simulink model "Template_v5_0_0_2026a_Original"  (R2026a)
settings: Solver=ode4  StopTime=tsim  FixedStep=baseRate  RelTol=1e-6  AbsTol=1e-6
undefined symbols (not defined in the file or in its folder): baseRate, dataRate, DiscIntNeverNeededParam, F_thrusters_BLACK, F_thrusters_BLUE, F_thrusters_RED, home_states_BLACK, home_states_BLUE, home_states_RED, IBLACK, IBLUE, init_states_BLACK, init_states_BLUE, init_states_RED, IRED, K_BLACK, K_BLUE, K_RED, labConsoleIP, mBLACK, mBLUE, mRED, Phase0_End, Phase1_End, Phase2_End, Phase3_End, Phase3_SubPhase1_End, Phase3_SubPhase2_End, Phase3_SubPhase3_End, Phase3_SubPhase4_End, Phase4_End, Phase5_End, platformSelection, PWMFreq, serverRate, simMode, tableDamping_BLACK, tableDamping_BLUE, tableDamping_RED, tableSlope, thrust_decay_BLACK, thrust_decay_BLUE, thrust_decay_RED, thruster_dist2CG_BLACK, thruster_dist2CG_BLUE, thruster_dist2CG_RED, xLength, yLength
libraries: simulink x18, dspinverses x3, nvidiaCommlib x1
(part 1 of 7)
settings Model: Creator=SPOT  LastModifiedBy=alexandercrain
settings OptimizationCC: MaxStackSize=200000
settings HardwareCC: ProdBitPerLong=64.0  ProdLargestAtomicInteger=LongLong  ProdLargestAtomicFloat=Double  ProdHWDeviceType=ARM Compatible->ARM Cortex-A (64-bit)
settings RTWCC: SystemTargetFile=ert.tlc  HardwareBoard=NVIDIA Jetson  TLCOptions="-aInlineSetEventsForThisBaseRateFcn=TLC_FALSE -aSuppressMultiTaskScheduler=TLC_FALSE  -aRateBasedStepFcn=0"  TargetLang=C++  Description=Embedded Coder
settings ERTTargetCC: ExtModeTransport=2.0  DynamicArrayContainerType=coder::array  SupportContinuousTime=on  SupportVariableSizeSignals=on
settings SimscapeCC: SimscapeNominalValues="[{\"value\":\"1\",\"unit\":\"A\"},{\"value\":\"1\",\"unit\":\"bar\"},{\"value\":\"1\",\"unit\":\"cm^2\"},{\"value\":\"1\",\"unit\":\"cm^3/s\"},{\"value\":\"1\",\"unit\":\"kJ/kg\"},{\"value\":\"1\",\"unit\":\"kW\"},{\"value\":\"1\",\"unit\":\"l\"},{\"value\":\"1\",\"unit\":\"N\"},{\"value\":\"1\",\"unit\":\"N*m\"},{\"value\":\"1\",\"unit\":\"V\"}]"  SimscapeLogType=none  SimscapeLogDataHistory=5000.0

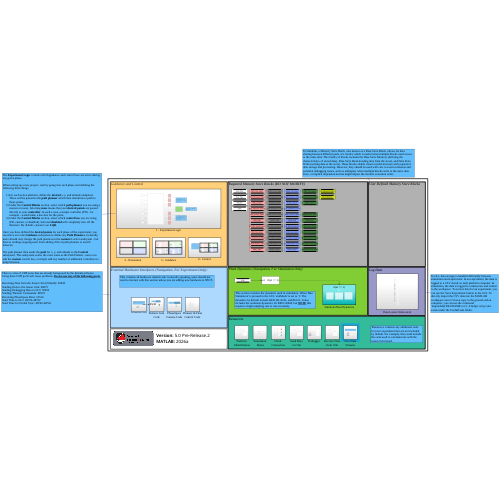
[thumbnail: Simulink's stored preview of the top-level diagram]
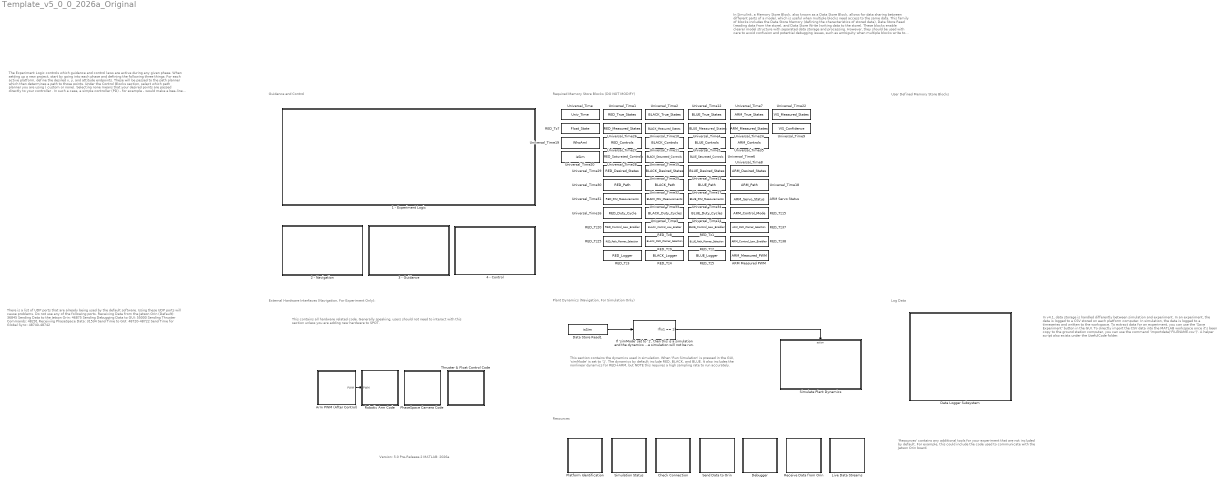
== system Template_v5_0_0_2026a_Original ==
  note: Version: 5.0 Pre-Release.2
      | MATLAB: 2026a
  note: Required Memory Store Blocks (DO NOT MODIFY)
  note: In Simulink, a Memory Store Block, also known as a Data Store Block, allows for data sharing between different parts of a model, which is useful when multiple blocks need access to the same data. This family of blocks includes the Data Store Memory (defining the characteristics of stored data), Data Store Read (reading data from the store), and Data Store Write (writing data to the store). These blocks enable clearer model structure with separated data storage and processing. However, they should be used with care to avoid confusion and potential debugging issues, such as ambiguity when multiple blocks write to the same data store, or implicit dependencies that might impact the model's execution order.
  note: User Defined Memory Store Blocks
  note: Log Data
  note: In v4.1, data storage is handled differently between simulation and experiment. In an experiment, the data is logged to a CSV stored on each platform computer. In simulation, the data is logged to a timeseries and written to the workspace. To extract data for an experiment, you can use the 'Save Experiment' button in the GUI. To directly import the CSV data into the MATLAB workspace once it's been copy to the ground station computer, you can use the command 'importdata('FILENAME.csv')'. A helper script also exists under the UsefulCode folder.
  note: Resources
  note: 'Resources' contains any additional tools for your experiment that are not included by default. For example, this could include the code used to communicate with the Jetson Orin board.
  note: Plant Dynamics (Navigation, For Simulation Only)
  note: This section contains the dynamics used in simulation. When 'Run Simulation' is pressed in the GUI, 'simMode' is set to '1'. The dynamics by default include RED, BLACK, and BLUE. It also includes the nonlinear dynamics for RED+ARM, but NOTE this requires a high sampling rate to run accurately.
  note: External Hardware Interfaces (Navigation, For Experiment Only):
  note: This contains all hardware related code. Generally speaking, users should not need to interact with this section unless you are adding new hardware to SPOT.
  note: Guidance and Control
  note: The Experiment Logic controls which guidance and control laws are active during any given phase.
      |
      | When setting up a new project, start by going into each phase and defining the following three things:
      |
      | For each active platform, define the desired x, y, and attitude endpoints. These will be passed to the path planner which then determines a path to those points.
      | Under the Control Blocks section, select which path planner you are using ( custom or none). Selecting none means that your desired points are passed directly to your controller . In such a case, a simple controller (PD) - for example - would make a bee-line for the point.
      | Under the Control Blocks section, select which control law you are using (PD, custom, or disabled). Selected disabled will completely turn off the thrusters. By default, custom is an LQR .
      |
      | Once you have defined the desired points for each phase of the experiment, you can move on to the Guidance subsystem to define any Path Planners. Generally, users should only change the path planners in the custom if-action subsytem - but there is nothing stopping users from adding 100s of path planners to switch between.
      |
      | The path planner then sends the path for x, y, and attitude to the Control subsystem. This subsystem works the exact same as the Path Planner - users can edit the custom control law, or simply add any number of additional controllers to jump between.
  note: There is a list of UDP ports that are already being used by the default software. Using these UDP ports will cause problems. Do not use any of the following ports.
      |
      | Receiving Data from the Jetson Orin (Default): 36845
      | Sending Data to the Jetson Orin: 46875
      | Sending Debugging Data to GUI: 55000
      | Sending Thruster Commands: 48291
      | Receiving PhaseSpace Data: 31534
      | Send Time to GUI: 48720-48722
      | Send Time for Global Sync: 48740-48742
  1 - Experiment Logic : Subsystem  Priority=30  TreatAsAtomicUnit=on
  2 - Navigation : Subsystem  Priority=40  TreatAsAtomicUnit=on
  3 - Guidance : Subsystem  Priority=40  TreatAsAtomicUnit=on
  4 - Control : Subsystem  Priority=50  TreatAsAtomicUnit=on
  ARM Measured PWM : DataStoreMemory  Description=ARM_Measured_PWM: the PWM each arm servo applies (its Present PWM, 885 = 100 % of the supply), written each step by the Dynamixel Arm (PWM) block on the hardware and by the RED + ARM Plant in simulation.  DataStoreName=ARM_Measured_PWM  WriteAfterWriteMsg=warning  InitialValue=[0;0;0]  ShowAdditionalParam=off
  ARM Servo Status : DataStoreMemory  Description="ARM_Controls: The simulated plant reads it at the start of each step, like the measurements, before the thruster code writes this step's command: the previous command acts for one step. (A loop through data stores needs one such step; with the plant first, the controllers get this step's measurements, as in experiments.) Before the first write, its initial value. (so its \"read before write\" and \"write after read\" checks are off)."  DataStoreName=ARM_Servo_Status  WriteAfterWriteMsg=warning  InitialValue=zeros(5,1)  ShowAdditionalParam=off
  Arm PWM (After Control) : Subsystem  Priority=61  TreatAsAtomicUnit=on
  Check Connection : Subsystem  Priority=71  TreatAsAtomicUnit=on
  Data Logger Subsystem : Subsystem  Priority=80  TreatAsAtomicUnit=on
  Data Store Read1 : DataStoreRead  Priority=24  DataStoreName=isSim  IndexOptions=Index vector (dialog)  Indices=1  OutputSizes=1
  Debugger : Subsystem  Priority=72  TreatAsAtomicUnit=on
  "If 'simMode' set to '1', then this is a simulation and the dynamics will be simulated. Otherwise, this is an experiment, and the simulation will not be run." : If  Priority=25  IfExpression=u1 == 1  ShowElse=off
  Live Data Streams : Subsystem  Priority=73  TreatAsAtomicUnit=on
  PhaseSpace Camera Code : Subsystem  Priority=20  TreatAsAtomicUnit=on
  Platform Identification : Subsystem  Priority=10  TreatAsAtomicUnit=on
  RED_Tz1 : DataStoreMemory  DataStoreName=BLUE_Control_Law_Enabler  ReadBeforeWriteMsg=warning  WriteAfterWriteMsg=warning  WriteAfterReadMsg=warning  ShowAdditionalParam=off
  RED_Tz15 : DataStoreMemory  DataStoreName=ARM_Control_Mode  WriteAfterWriteMsg=warning  ShowAdditionalParam=off
  RED_Tz2 : DataStoreMemory  DataStoreName=BLUE_Path_Planner_Selection  ReadBeforeWriteMsg=warning  WriteAfterWriteMsg=warning  WriteAfterReadMsg=warning  ShowAdditionalParam=off
  RED_Tz20 : DataStoreMemory  DataStoreName=RED_Control_Law_Enabler  ReadBeforeWriteMsg=warning  WriteAfterWriteMsg=warning  WriteAfterReadMsg=warning  ShowAdditionalParam=off
  RED_Tz25 : DataStoreMemory  DataStoreName=RED_Path_Planner_Selection  ReadBeforeWriteMsg=warning  WriteAfterWriteMsg=warning  WriteAfterReadMsg=warning  ShowAdditionalParam=off
  RED_Tz3 : DataStoreMemory  DataStoreName=RED_Logger  ReadBeforeWriteMsg=warning  WriteAfterWriteMsg=warning  WriteAfterReadMsg=warning  ShowAdditionalParam=off
  RED_Tz37 : DataStoreMemory  DataStoreName=ARM_Path_Planner_Selection  ReadBeforeWriteMsg=warning  WriteAfterWriteMsg=warning  WriteAfterReadMsg=warning  ShowAdditionalParam=off
  RED_Tz38 : DataStoreMemory  DataStoreName=ARM_Control_Law_Enabler  ReadBeforeWriteMsg=warning  WriteAfterWriteMsg=warning  WriteAfterReadMsg=warning  ShowAdditionalParam=off
  RED_Tz4 : DataStoreMemory  DataStoreName=BLACK_Logger  ReadBeforeWriteMsg=warning  WriteAfterWriteMsg=warning  WriteAfterReadMsg=warning  ShowAdditionalParam=off
  RED_Tz5 : DataStoreMemory  DataStoreName=BLUE_Logger  ReadBeforeWriteMsg=warning  WriteAfterWriteMsg=warning  WriteAfterReadMsg=warning  ShowAdditionalParam=off
  RED_Tz7 : DataStoreMemory  Description=Read-before-write and write-after-read checks off: Simulate Plant Dynamics (priority 25) reads it to apply the table's slope only while the platforms float, a step before 1 - Experiment Logic (30) writes it.  DataStoreName=Float_State  WriteAfterWriteMsg=warning  ShowAdditionalParam=off
  RED_Tz8 : DataStoreMemory  DataStoreName=BLACK_Control_Law_Enabler  ReadBeforeWriteMsg=warning  WriteAfterWriteMsg=warning  WriteAfterReadMsg=warning  ShowAdditionalParam=off
  RED_Tz9 : DataStoreMemory  DataStoreName=BLACK_Path_Planner_Selection  ReadBeforeWriteMsg=warning  WriteAfterWriteMsg=warning  WriteAfterReadMsg=warning  ShowAdditionalParam=off
  Receive Data from Orin : Subsystem  Priority=22  TreatAsAtomicUnit=on
  Robotic Arm Code : Subsystem  Priority=21  TreatAsAtomicUnit=on
  Send Data to Orin : Subsystem  Priority=70  TreatAsAtomicUnit=on
  Simulate Plant Dynamics : Subsystem  TreatAsAtomicUnit=on
  Simulation Status : Subsystem  Priority=5  TreatAsAtomicUnit=on
  Thruster & Float Control Code : Subsystem  Priority=60  TreatAsAtomicUnit=on  SystemSampleTime=baseRate
  Universal_Time : DataStoreMemory  DataStoreName=Univ_Time  ReadBeforeWriteMsg=warning  WriteAfterWriteMsg=warning  WriteAfterReadMsg=warning  ShowAdditionalParam=off
  Universal_Time1 : DataStoreMemory  DataStoreName=RED_True_States  ReadBeforeWriteMsg=warning  WriteAfterWriteMsg=warning  WriteAfterReadMsg=warning  InitialValue=[0;0;0;0;0;0;0;0;0]  ShowAdditionalParam=off
  Universal_Time10 : DataStoreMemory  DataStoreName=BLACK_Measured_States  ReadBeforeWriteMsg=warning  WriteAfterWriteMsg=warning  WriteAfterReadMsg=warning  InitialValue=[0;0;0;0;0;0;0;0;0]  ShowAdditionalParam=off
  Universal_Time11 : DataStoreMemory  DataStoreName=BLACK_Controls  ReadBeforeWriteMsg=warning  WriteAfterWriteMsg=warning  WriteAfterReadMsg=warning  InitialValue=[0;0;0]  ShowAdditionalParam=off
  Universal_Time12 : DataStoreMemory  DataStoreName=BLUE_True_States  ReadBeforeWriteMsg=warning  WriteAfterWriteMsg=warning  WriteAfterReadMsg=warning  InitialValue=[0;0;0;0;0;0;0;0;0]  ShowAdditionalParam=off
  Universal_Time13 : DataStoreMemory  Description="BLUE_Desired_States: Written only in the phases that use it; it keeps its value in between (before the first write, its initial value). (so its \"read before write\" check is off)."  DataStoreName=BLUE_Desired_States  WriteAfterWriteMsg=warning  WriteAfterReadMsg=warning  InitialValue=[0;0;0]  ShowAdditionalParam=off
  Universal_Time14 : DataStoreMemory  DataStoreName=BLUE_Duty_Cycles  ReadBeforeWriteMsg=warning  WriteAfterWriteMsg=warning  WriteAfterReadMsg=warning  InitialValue=[0;0;0;0;0;0;0;0]  ShowAdditionalParam=off
  Universal_Time15 : DataStoreMemory  Description="BLACK_Saturated_Controls: The simulated plant reads it at the start of each step, like the measurements, before the thruster code writes this step's command: the previous command acts for one step. (A loop through data stores needs one such step; with the plant first, the controllers get this step's measurements, as in experiments.) Before the first write, its initial value. (so its \"read before write\" and \"write after read\" checks are off)."  DataStoreName=BLACK_Saturated_Controls  WriteAfterWriteMsg=warning  InitialValue=[0;0;0]  ShowAdditionalParam=off
  Universal_Time16 : DataStoreMemory  DataStoreName=RED_Duty_Cycle  ReadBeforeWriteMsg=warning  WriteAfterWriteMsg=warning  WriteAfterReadMsg=warning  InitialValue=[0;0;0;0;0;0;0;0]  ShowAdditionalParam=off
  Universal_Time17 : DataStoreMemory  DataStoreName=BLUE_Path  ReadBeforeWriteMsg=warning  WriteAfterWriteMsg=warning  WriteAfterReadMsg=warning  InitialValue=[0;0;0]  ShowAdditionalParam=off
  Universal_Time18 : DataStoreMemory  DataStoreName=ARM_Path  ReadBeforeWriteMsg=warning  WriteAfterWriteMsg=warning  WriteAfterReadMsg=warning  InitialValue=[0;0;0]  ShowAdditionalParam=off
  Universal_Time19 : DataStoreMemory  Description="WhoAmI: Written only in experiments (or, for the arm, when the arm is simulated); otherwise it keeps its initial value. (so its \"read before write\" check is off)."  DataStoreName=WhoAmI  WriteAfterWriteMsg=warning  WriteAfterReadMsg=warning  ShowAdditionalParam=off
  Universal_Time2 : DataStoreMemory  DataStoreName=BLACK_True_States  ReadBeforeWriteMsg=warning  WriteAfterWriteMsg=warning  WriteAfterReadMsg=warning  InitialValue=[0;0;0;0;0;0;0;0;0]  ShowAdditionalParam=off
  Universal_Time20 : DataStoreMemory  DataStoreName=isSim  ReadBeforeWriteMsg=warning  WriteAfterWriteMsg=warning  WriteAfterReadMsg=warning  ShowAdditionalParam=off
  Universal_Time22 : DataStoreMemory  Description="VIS_Measured_States: Written only in experiments (or, for the arm, when the arm is simulated); otherwise it keeps its initial value. (so its \"read before write\" check is off)."  DataStoreName=VIS_Measured_States  WriteAfterWriteMsg=warning  WriteAfterReadMsg=warning  InitialValue=[0;0;0]  ShowAdditionalParam=off
  Universal_Time24 : DataStoreMemory  Description="ARM_Measured_States: Written only in experiments (or, for the arm, when the arm is simulated); otherwise it keeps its initial value. (so its \"read before write\" check is off)."  DataStoreName=ARM_Measured_States  WriteAfterWriteMsg=warning  WriteAfterReadMsg=warning  InitialValue=[0;0;0;0;0;0]  ShowAdditionalParam=off
  Universal_Time25 : DataStoreMemory  Description="BLACK_Desired_States: Written only in the phases that use it; it keeps its value in between (before the first write, its initial value). (so its \"read before write\" check is off)."  DataStoreName=BLACK_Desired_States  WriteAfterWriteMsg=warning  WriteAfterReadMsg=warning  InitialValue=[0;0;0]  ShowAdditionalParam=off
  Universal_Time26 : DataStoreMemory  DataStoreName=RED_Measured_States  ReadBeforeWriteMsg=warning  WriteAfterWriteMsg=warning  WriteAfterReadMsg=warning  InitialValue=[0;0;0;0;0;0;0;0;0]  ShowAdditionalParam=off
  Universal_Time27 : DataStoreMemory  DataStoreName=RED_Controls  ReadBeforeWriteMsg=warning  WriteAfterWriteMsg=warning  WriteAfterReadMsg=warning  InitialValue=[0;0;0]  ShowAdditionalParam=off
  Universal_Time28 : DataStoreMemory  Description="RED_Saturated_Controls: The simulated plant reads it at the start of each step, like the measurements, before the thruster code writes this step's command: the previous command acts for one step. (A loop through data stores needs one such step; with the plant first, the controllers get this step's measurements, as in experiments.) Before the first write, its initial value. (so its \"read before write\" and \"write after read\" checks are off)."  DataStoreName=RED_Saturated_Controls  WriteAfterWriteMsg=warning  InitialValue=[0;0;0]  ShowAdditionalParam=off
  Universal_Time29 : DataStoreMemory  Description="RED_Desired_States: Written only in the phases that use it; it keeps its value in between (before the first write, its initial value). (so its \"read before write\" check is off)."  DataStoreName=RED_Desired_States  WriteAfterWriteMsg=warning  WriteAfterReadMsg=warning  InitialValue=[0;0;0]  ShowAdditionalParam=off
  Universal_Time3 : DataStoreMemory  DataStoreName=BLACK_Duty_Cycles  ReadBeforeWriteMsg=warning  WriteAfterWriteMsg=warning  WriteAfterReadMsg=warning  InitialValue=[0;0;0;0;0;0;0;0]  ShowAdditionalParam=off
  Universal_Time30 : DataStoreMemory  DataStoreName=RED_Path  ReadBeforeWriteMsg=warning  WriteAfterWriteMsg=warning  WriteAfterReadMsg=warning  InitialValue=[0;0;0]  ShowAdditionalParam=off
  Universal_Time31 : DataStoreMemory  Description="RED_IMU_Measurements: Nothing writes it yet: a placeholder for IMU data, logged as its initial value. (so its \"read before write\" check is off)."  DataStoreName=RED_IMU_Measurements  WriteAfterWriteMsg=warning  WriteAfterReadMsg=warning  InitialValue=[0;0;0]  ShowAdditionalParam=off
  Universal_Time32 : DataStoreMemory  DataStoreName=BLACK_Path  ReadBeforeWriteMsg=warning  WriteAfterWriteMsg=warning  WriteAfterReadMsg=warning  InitialValue=[0;0;0]  ShowAdditionalParam=off
  Universal_Time33 : DataStoreMemory  Description="BLACK_IMU_Measurements: Nothing writes it yet: a placeholder for IMU data, logged as its initial value. (so its \"read before write\" check is off)."  DataStoreName=BLACK_IMU_Measurements  WriteAfterWriteMsg=warning  WriteAfterReadMsg=warning  InitialValue=[0;0;0]  ShowAdditionalParam=off
  Universal_Time34 : DataStoreMemory  Description="BLUE_IMU_Measurements: Nothing writes it yet: a placeholder for IMU data, logged as its initial value. (so its \"read before write\" check is off)."  DataStoreName=BLUE_IMU_Measurements  WriteAfterWriteMsg=warning  WriteAfterReadMsg=warning  InitialValue=[0;0;0]  ShowAdditionalParam=off
  Universal_Time35 : DataStoreMemory  Description="ARM_Controls: The simulated plant reads it at the start of each step, like the measurements, before the thruster code writes this step's command: the previous command acts for one step. (A loop through data stores needs one such step; with the plant first, the controllers get this step's measurements, as in experiments.) Before the first write, its initial value. (so its \"read before write\" and \"write after read\" checks are off)."  DataStoreName=ARM_Controls  WriteAfterWriteMsg=warning  InitialValue=[0;0;0]  ShowAdditionalParam=off
  Universal_Time4 : DataStoreMemory  DataStoreName=BLUE_Measured_States  ReadBeforeWriteMsg=warning  WriteAfterWriteMsg=warning  WriteAfterReadMsg=warning  InitialValue=[0;0;0;0;0;0;0;0;0]  ShowAdditionalParam=off
  Universal_Time5 : DataStoreMemory  DataStoreName=BLUE_Controls  ReadBeforeWriteMsg=warning  WriteAfterWriteMsg=warning  WriteAfterReadMsg=warning  InitialValue=[0;0;0]  ShowAdditionalParam=off
  Universal_Time6 : DataStoreMemory  Description="BLUE_Saturated_Controls: The simulated plant reads it at the start of each step, like the measurements, before the thruster code writes this step's command: the previous command acts for one step. (A loop through data stores needs one such step; with the plant first, the controllers get this step's measurements, as in experiments.) Before the first write, its initial value. (so its \"read before write\" and \"write after read\" checks are off)."  DataStoreName=BLUE_Saturated_Controls  WriteAfterWriteMsg=warning  InitialValue=[0;0;0]  ShowAdditionalParam=off
  Universal_Time7 : DataStoreMemory  DataStoreName=ARM_True_States  ReadBeforeWriteMsg=warning  WriteAfterWriteMsg=warning  WriteAfterReadMsg=warning  InitialValue=[0;0;0;0;0;0]  ShowAdditionalParam=off
  Universal_Time8 : DataStoreMemory  Description="ARM_Desired_States: Written only in the phases that use it; it keeps its value in between (before the first write, its initial value). (so its \"read before write\" check is off)."  DataStoreName=ARM_Desired_States  WriteAfterWriteMsg=warning  WriteAfterReadMsg=warning  InitialValue=[0;0;0]  ShowAdditionalParam=off
  Universal_Time9 : DataStoreMemory  Description="VIS_Confidence: Written only in experiments (or, for the arm, when the arm is simulated); otherwise it keeps its initial value. (so its \"read before write\" check is off)."  DataStoreName=VIS_Confidence  WriteAfterWriteMsg=warning  WriteAfterReadMsg=warning  ShowAdditionalParam=off
  wires:
  Data Store Read1/1 -> "If 'simMode' set to '1', then this is a simulation and the dynamics will be simulated. Otherwise, this is an experiment, and the simulation will not be run."/1
  "If 'simMode' set to '1', then this is a simulation and the dynamics will be simulated. Otherwise, this is an experiment, and the simulation will not be run."/1 -> Simulate Plant Dynamics/Action
  Arm PWM (After Control)/1(PWM) -> Robotic Arm Code/1(PWM)

== system Template_v5_0_0_2026a_Original/1 - Experiment Logic ==
  note: As a general rule, users should not need to edit these phases. If the initial position must be changed, this change should be made in the GUI.
  note: As a general rule, users should not need to edit these phases. If the home position must be changed, this change should be made in the GUI.
  note: Users should only be editing the sub-systems under Phase #3: Experiment
  Constant : Constant  Value=Phase1_End  SampleTime=-1
  Constant1 : Constant  Value=Phase2_End  SampleTime=-1
  Constant2 : Constant  Value=Phase3_End  SampleTime=-1
  Constant3 : Constant  Value=Phase4_End  SampleTime=-1
  Constant4 : Constant  Value=Phase0_End  SampleTime=-1
  Constant6 : Constant  Value=Phase5_End  SampleTime=-1
  Phase #0: Synchronization : Subsystem  TreatAsAtomicUnit=on
  "Phase #1: Start Floating " : Subsystem  TreatAsAtomicUnit=on
  Phase #2: Initial Position : Subsystem  TreatAsAtomicUnit=on
  Phase #3: Experiment : Subsystem  TreatAsAtomicUnit=on
  Phase #4: Return Home : Subsystem  TreatAsAtomicUnit=on
  Phase #5: Hold Home : Subsystem  TreatAsAtomicUnit=on
  Phase #6: Clean Shutdown : Subsystem  TreatAsAtomicUnit=on
  Separate Phases : If  NumInputs=7  IfExpression=u1 < u2  ElseIfExpressions=(u1 < u3 & u1 >= u2),(u1 < u4 & u1 >= u3), (u1 < u5 & u1 >= u4),(u1 < u6 & u1 >= u5), (u1 < u7 & u1 >= u6) ,(u1 >= u7)  ShowElse=off
  Universal_Time25 : DataStoreRead  DataStoreName=Univ_Time  IndexOptions=Index vector (dialog)  Indices=1  OutputSizes=1
  wires:
  Separate Phases/2 -> "Phase #1: Start Floating "/Action
  Universal_Time25/1 -> Separate Phases/1
  Separate Phases/4 -> Phase #3: Experiment/Action
  Constant2/1 -> Separate Phases/5
  Separate Phases/7 -> Phase #6: Clean Shutdown/Action
  Constant6/1 -> Separate Phases/7
  Separate Phases/6 -> Phase #5: Hold Home/Action
  Separate Phases/1 -> Phase #0: Synchronization/Action
  Constant4/1 -> Separate Phases/2
  Constant/1 -> Separate Phases/3
  Separate Phases/5 -> Phase #4: Return Home/Action
  Separate Phases/3 -> Phase #2: Initial Position/Action
  Constant3/1 -> Separate Phases/6
  Constant1/1 -> Separate Phases/4

== system Template_v5_0_0_2026a_Original/2 - Navigation ==
  note: Navigation Filters (RED)
  note: Navigation Filters (Robotic Manipulator)
  note: Navigation Filters (BLUE)
  note: Navigation Filters (BLACK)

== system Template_v5_0_0_2026a_Original/3 - Guidance ==
  note: Path Planners (RED)
  note: Path Planners (Robotic Manipulator)
  note: Path Planners (BLUE)
  note: Path Planners (BLACK)
  Custom PPL (ARM) : Subsystem  TreatAsAtomicUnit=on
  Custom PPL (BLACK) : Subsystem  TreatAsAtomicUnit=on
  Custom PPL (BLUE) : Subsystem  TreatAsAtomicUnit=on
  Custom PPL (RED) : Subsystem  TreatAsAtomicUnit=on
  Data Store Read : DataStoreRead  DataStoreName=RED_Path_Planner_Selection  IndexOptions=Index vector (dialog)  Indices=1  OutputSizes=1
  Data Store Read1 : DataStoreRead  DataStoreName=BLACK_Path_Planner_Selection  IndexOptions=Index vector (dialog)  Indices=1  OutputSizes=1
  Data Store Read2 : DataStoreRead  DataStoreName=ARM_Path_Planner_Selection  IndexOptions=Index vector (dialog)  Indices=1  OutputSizes=1
  Data Store Read3 : DataStoreRead  DataStoreName=BLUE_Path_Planner_Selection  IndexOptions=Index vector (dialog)  Indices=1  OutputSizes=1
  Data Store Write : DataStoreWrite  DataStoreName=RED_Path  IndexOptions=Index vector (dialog)  Indices=1  OutputSizes=1
  Data Store Write3 : DataStoreWrite  DataStoreName=BLACK_Path  IndexOptions=Index vector (dialog)  Indices=1  OutputSizes=1
  Data Store Write6 : DataStoreWrite  DataStoreName=BLUE_Path  IndexOptions=Index vector (dialog)  Indices=1  OutputSizes=1
  Data Store Write9 : DataStoreWrite  DataStoreName=ARM_Path  IndexOptions=Index vector (dialog)  Indices=1  OutputSizes=1
  Disable PPL (ARM) : Subsystem  TreatAsAtomicUnit=on
  Disable PPL (BLACK) : Subsystem  TreatAsAtomicUnit=on
  Disable PPL (BLUE) : Subsystem  TreatAsAtomicUnit=on
  Disable PPL (RED) : Subsystem  TreatAsAtomicUnit=on
  If : If  IfExpression=u1 == 1
  If1 : If  IfExpression=u1 == 1
  If2 : If  IfExpression=u1 == 2
  If3 : If  IfExpression=u1 == 2
  Merge{,1..3} (4 alike) : Merge
  wires:
  Data Store Read/1 -> If/1
  Merge/1 -> Data Store Write/1
  If/2 -> Disable PPL (RED)/Action
  If/1 -> Custom PPL (RED)/Action
  Disable PPL (RED)/1(Path) -> Merge/2
  Data Store Read1/1 -> If1/1
  Disable PPL (BLACK)/1(Path) -> Merge1/2
  If1/2 -> Disable PPL (BLACK)/Action
  If1/1 -> Custom PPL (BLACK)/Action
  Merge1/1 -> Data Store Write3/1
  Merge2/1 -> Data Store Write6/1
  Disable PPL (BLUE)/1(Path) -> Merge2/2
  If2/2 -> Disable PPL (BLUE)/Action
  If2/1 -> Custom PPL (BLUE)/Action
  Data Store Read3/1 -> If2/1
  If3/1 -> Custom PPL (ARM)/Action
  Merge3/1 -> Data Store Write9/1
  Disable PPL (ARM)/1(Path) -> Merge3/2
  Data Store Read2/1 -> If3/1
  If3/2 -> Disable PPL (ARM)/Action
  Custom PPL (BLUE)/1(Path) -> Merge2/1
  Custom PPL (ARM)/1(Path) -> Merge3/1
  Custom PPL (RED)/1(Path) -> Merge/1
  Custom PPL (BLACK)/1(Path) -> Merge1/1

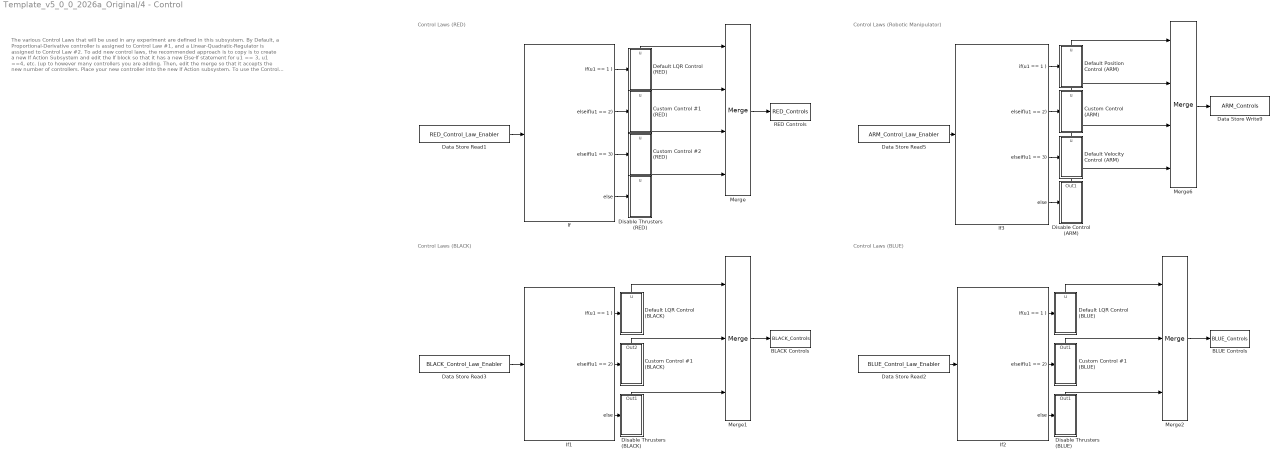
== system Template_v5_0_0_2026a_Original/4 - Control ==
  note: Control Laws (RED)
  note: Control Laws (Robotic Manipulator)
  note: Control Laws (BLUE)
  note: Control Laws (BLACK)
  note: The various Control Laws that will be used in any experiment are defined in this subsystem. By Default, a Proportional-Derivative controller is assigned to Control Law #1, and a Linear-Quadratic-Regulator is assigned to Control Law #2.
      |
      | To add new control laws, the recommended approach is to copy is to create a new If Action Subsystem and edit the If block so that it has a new Else-If statement for u1 == 3, u1 ==4, etc. (up to however many controllers you are adding.
      |
      | Then, edit the merge so that it accepts the new number of controllers. Place your new controller into the new If Action subsystem.
      |
      | To use the Control Law, in the Experiment Phases change the input to the relevant Control Law Enabler to match the controller you want to use - in this example, that would be #3.
      |
      | The RED control law section on this page has been configured to have one extra If Action subsystem to demonstrate how this should look when it is properly set up.
      |
      | Note, any controller number that is not assigned (in this case, any number other then 1, 2, and 3) will disable the thrusters due to the Else statement.
  BLACK Controls : DataStoreWrite  DataStoreName=BLACK_Controls  IndexOptions=Index vector (dialog)  Indices=1  OutputSizes=1
  BLUE Controls : DataStoreWrite  DataStoreName=BLUE_Controls  IndexOptions=Index vector (dialog)  Indices=1  OutputSizes=1
  Custom Control #1 (BLACK) : Subsystem  TreatAsAtomicUnit=on
  Custom Control #1 (BLUE) : Subsystem  TreatAsAtomicUnit=on
  Custom Control #1 (RED) : Subsystem  TreatAsAtomicUnit=on
  Custom Control #2 (RED) : Subsystem  TreatAsAtomicUnit=on
  Custom Control (ARM) : Subsystem  TreatAsAtomicUnit=on
  Data Store Read1 : DataStoreRead  DataStoreName=RED_Control_Law_Enabler  IndexOptions=Index vector (dialog)  Indices=1  OutputSizes=1
  Data Store Read2 : DataStoreRead  DataStoreName=BLUE_Control_Law_Enabler  IndexOptions=Index vector (dialog)  Indices=1  OutputSizes=1
  Data Store Read3 : DataStoreRead  DataStoreName=BLACK_Control_Law_Enabler  IndexOptions=Index vector (dialog)  Indices=1  OutputSizes=1
  Data Store Read5 : DataStoreRead  DataStoreName=ARM_Control_Law_Enabler  IndexOptions=Index vector (dialog)  Indices=1  OutputSizes=1
  Data Store Write9 : DataStoreWrite  DataStoreName=ARM_Controls  IndexOptions=Index vector (dialog)  Indices=1  OutputSizes=1
  Default LQR Control (BLACK) : Subsystem  TreatAsAtomicUnit=on
  Default LQR Control (BLUE) : Subsystem  TreatAsAtomicUnit=on
  Default LQR Control (RED) : Subsystem  TreatAsAtomicUnit=on
  Default Position Control (ARM) : Subsystem  TreatAsAtomicUnit=on
  Default Velocity Control (ARM) : Subsystem  TreatAsAtomicUnit=on
  Disable Control (ARM) : Subsystem  TreatAsAtomicUnit=on
  Disable Thrusters (BLACK) : Subsystem  TreatAsAtomicUnit=on
  Disable Thrusters (BLUE) : Subsystem  TreatAsAtomicUnit=on
  Disable Thrusters (RED) : Subsystem  TreatAsAtomicUnit=on
  If : If  IfExpression=u1 == 1  ElseIfExpressions=u1 == 2, u1 == 3
  If1 : If  IfExpression=u1 == 1  ElseIfExpressions=u1 == 2
  If2 : If  IfExpression=u1 == 1  ElseIfExpressions=u1 == 2
  If3 : If  IfExpression=u1 == 1  ElseIfExpressions=u1 == 2, u1 == 3
  Merge : Merge  Inputs=4
  Merge1 : Merge  Inputs=3
  Merge2 : Merge  Inputs=3
  Merge6 : Merge  Inputs=4
  RED Controls : DataStoreWrite  DataStoreName=RED_Controls  IndexOptions=Index vector (dialog)  Indices=1  OutputSizes=1
  wires:
  Data Store Read1/1 -> If/1
  Merge/1 -> RED Controls/1
  If/4 -> Disable Thrusters (RED)/Action
  If/2 -> Custom Control #1 (RED)/Action
  If1/1 -> Default LQR Control (BLACK)/Action
  If1/2 -> Custom Control #1 (BLACK)/Action
  Merge1/1 -> BLACK Controls/1
  Data Store Read3/1 -> If1/1
  If1/3 -> Disable Thrusters (BLACK)/Action
  Data Store Read2/1 -> If2/1
  If2/3 -> Disable Thrusters (BLUE)/Action
  Merge2/1 -> BLUE Controls/1
  Default LQR Control (BLUE)/1(u) -> Merge2/1
  Custom Control #1 (BLUE)/1(Out1) -> Merge2/2
  Disable Thrusters (BLUE)/1(Out1) -> Merge2/3
  Disable Thrusters (BLACK)/1(Out1) -> Merge1/3
  Merge6/1 -> Data Store Write9/1
  Custom Control (ARM)/1(u) -> Merge6/2
  If3/1 -> Default Position Control (ARM)/Action
  If3/2 -> Custom Control (ARM)/Action
  Data Store Read5/1 -> If3/1
  Default Position Control (ARM)/1(u) -> Merge6/1
  Default LQR Control (BLACK)/1(u) -> Merge1/1
  Custom Control #1 (BLACK)/1(Out2) -> Merge1/2
  If/3 -> Custom Control #2 (RED)/Action
  Default LQR Control (RED)/1(u) -> Merge/1
  Custom Control #1 (RED)/1(u) -> Merge/2
  Custom Control #2 (RED)/1(u) -> Merge/3
  Disable Thrusters (RED)/1(u) -> Merge/4
  If/1 -> Default LQR Control (RED)/Action
  If2/2 -> Custom Control #1 (BLUE)/Action
  If2/1 -> Default LQR Control (BLUE)/Action
  If3/3 -> Default Velocity Control (ARM)/Action
  If3/4 -> Disable Control (ARM)/Action
  Disable Control (ARM)/1(Out1) -> Merge6/4
  Default Velocity Control (ARM)/1(u) -> Merge6/3

== system Template_v5_0_0_2026a_Original/Arm PWM (After Control) ==
  note: This step's ARM_Controls (joint PWM [885 = 100 %]), read after 4 - Control (priority 61), for the Dynamixel Arm (PWM) block in Robotic Arm Code: it reads the encoders at priority 21 and sends this PWM at the end of the step, so a command goes out in the step it was computed, as in the simulation.
  Data Store Read : DataStoreRead  DataStoreName=ARM_Controls  IndexOptions=Index vector (dialog)  Indices=1  OutputSizes=1
  PWM : Outport
  wires:
  Data Store Read/1 -> PWM/1

== system Template_v5_0_0_2026a_Original/Check Connection ==
  Change BLACK Behavior : Subsystem  TreatAsAtomicUnit=on
  Change BLUE Behavior : Subsystem  TreatAsAtomicUnit=on
  Change RED Behavior : Subsystem  TreatAsAtomicUnit=on
  Data Store Read : DataStoreRead  DataStoreName=WhoAmI  IndexOptions=Index vector (dialog)  Indices=1  OutputSizes=1
  Data Store Read1 : DataStoreRead  DataStoreName=isSim  IndexOptions=Index vector (dialog)  Indices=1  OutputSizes=1
  This IF block determines whether or not to run the BLACK sim/exp : If  NumInputs=2  IfExpression=u1 == 2 & u2 == 0  ShowElse=off
  This IF block determines whether or not to run the BLUE sim/exp : If  NumInputs=2  IfExpression=u1 == 3 & u2 == 0  ShowElse=off
  "This IF block determines whether or not to run the RED sim/exp " : If  NumInputs=2  IfExpression=u1 == 1 & u2 == 0  ShowElse=off
  wires:
  This IF block determines whether or not to run the BLACK sim/exp/1 -> Change BLACK Behavior/Action
  "This IF block determines whether or not to run the RED sim/exp "/1 -> Change RED Behavior/Action
  Data Store Read/1 -> This IF block determines whether or not to run the BLUE sim/exp/1, This IF block determines whether or not to run the BLACK sim/exp/1, "This IF block determines whether or not to run the RED sim/exp "/1
  This IF block determines whether or not to run the BLUE sim/exp/1 -> Change BLUE Behavior/Action
  Data Store Read1/1 -> This IF block determines whether or not to run the BLACK sim/exp/2, This IF block determines whether or not to run the BLUE sim/exp/2, "This IF block determines whether or not to run the RED sim/exp "/2

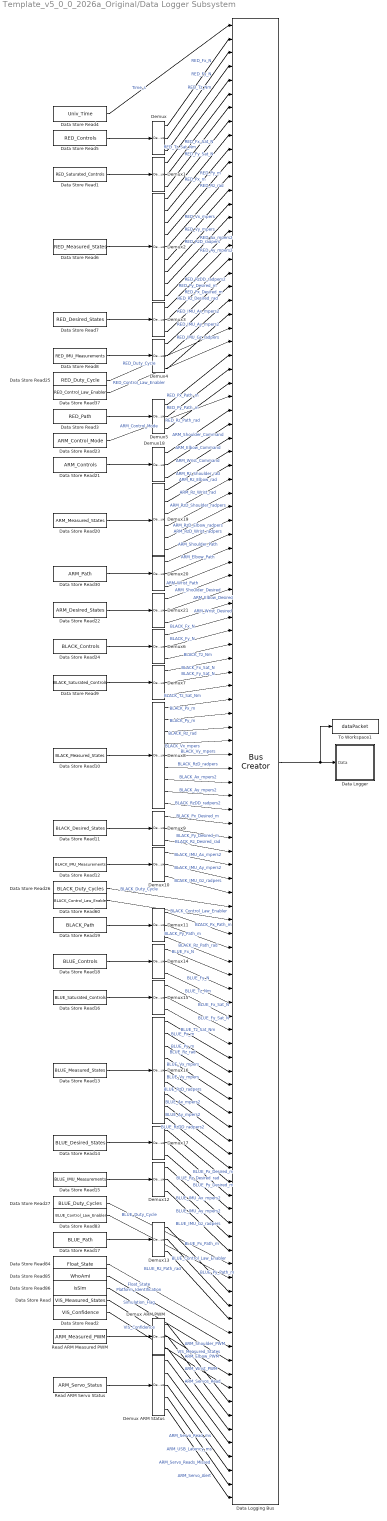
== system Template_v5_0_0_2026a_Original/Data Logger Subsystem ==
  Data Logger : Subsystem
  Data Logging Bus : BusCreator  Inputs=108
  Data Store Read : DataStoreRead  DataStoreName=VIS_Measured_States  IndexOptions=Index vector (dialog)  Indices=1  OutputSizes=1
  Data Store Read1 : DataStoreRead  DataStoreName=RED_Saturated_Controls  IndexOptions=Index vector (dialog)  Indices=1  OutputSizes=1
  Data Store Read10 : DataStoreRead  DataStoreName=BLACK_Measured_States  IndexOptions=Index vector (dialog)  Indices=1  OutputSizes=1
  Data Store Read11 : DataStoreRead  DataStoreName=BLACK_Desired_States  IndexOptions=Index vector (dialog)  Indices=1  OutputSizes=1
  Data Store Read12 : DataStoreRead  DataStoreName=BLACK_IMU_Measurements  IndexOptions=Index vector (dialog)  Indices=1  OutputSizes=1
  Data Store Read13 : DataStoreRead  DataStoreName=BLUE_Measured_States  IndexOptions=Index vector (dialog)  Indices=1  OutputSizes=1
  Data Store Read14 : DataStoreRead  DataStoreName=BLUE_Desired_States  IndexOptions=Index vector (dialog)  Indices=1  OutputSizes=1
  Data Store Read15 : DataStoreRead  DataStoreName=BLUE_IMU_Measurements  IndexOptions=Index vector (dialog)  Indices=1  OutputSizes=1
  Data Store Read16 : DataStoreRead  DataStoreName=BLUE_Saturated_Controls  IndexOptions=Index vector (dialog)  Indices=1  OutputSizes=1
  Data Store Read17 : DataStoreRead  DataStoreName=BLUE_Path  IndexOptions=Index vector (dialog)  Indices=1  OutputSizes=1
  Data Store Read18 : DataStoreRead  DataStoreName=BLUE_Controls  IndexOptions=Index vector (dialog)  Indices=1  OutputSizes=1
  Data Store Read19 : DataStoreRead  DataStoreName=BLACK_Path  IndexOptions=Index vector (dialog)  Indices=1  OutputSizes=1
  Data Store Read2 : DataStoreRead  DataStoreName=VIS_Confidence  IndexOptions=Index vector (dialog)  Indices=1  OutputSizes=1
  Data Store Read20 : DataStoreRead  DataStoreName=ARM_Measured_States  IndexOptions=Index vector (dialog)  Indices=1  OutputSizes=1
  Data Store Read21 : DataStoreRead  DataStoreName=ARM_Controls  IndexOptions=Index vector (dialog)  Indices=1  OutputSizes=1
  Data Store Read22 : DataStoreRead  DataStoreName=ARM_Desired_States  IndexOptions=Index vector (dialog)  Indices=1  OutputSizes=1
  Data Store Read23 : DataStoreRead  DataStoreName=ARM_Control_Mode  IndexOptions=Index vector (dialog)  Indices=1  OutputSizes=1
  Data Store Read24 : DataStoreRead  DataStoreName=BLACK_Controls  IndexOptions=Index vector (dialog)  Indices=1  OutputSizes=1
  Data Store Read25 : DataStoreRead  DataStoreName=RED_Duty_Cycle  IndexOptions=Index vector (dialog)  Indices=1  OutputSizes=1
  Data Store Read26 : DataStoreRead  DataStoreName=BLACK_Duty_Cycles  IndexOptions=Index vector (dialog)  Indices=1  OutputSizes=1
  Data Store Read27 : DataStoreRead  DataStoreName=BLUE_Duty_Cycles  IndexOptions=Index vector (dialog)  Indices=1  OutputSizes=1
  Data Store Read3 : DataStoreRead  DataStoreName=RED_Path  IndexOptions=Index vector (dialog)  Indices=1  OutputSizes=1
  Data Store Read30 : DataStoreRead  DataStoreName=ARM_Path  IndexOptions=Index vector (dialog)  Indices=1  OutputSizes=1
  Data Store Read37 : DataStoreRead  DataStoreName=RED_Control_Law_Enabler  IndexOptions=Index vector (dialog)  Indices=1  OutputSizes=1
  Data Store Read4 : DataStoreRead  DataStoreName=Univ_Time  IndexOptions=Index vector (dialog)  Indices=1  OutputSizes=1
  Data Store Read5 : DataStoreRead  DataStoreName=RED_Controls  IndexOptions=Index vector (dialog)  Indices=1  OutputSizes=1
  Data Store Read6 : DataStoreRead  DataStoreName=RED_Measured_States  IndexOptions=Index vector (dialog)  Indices=1  OutputSizes=1
  Data Store Read60 : DataStoreRead  DataStoreName=BLACK_Control_Law_Enabler  IndexOptions=Index vector (dialog)  Indices=1  OutputSizes=1
  Data Store Read7 : DataStoreRead  DataStoreName=RED_Desired_States  IndexOptions=Index vector (dialog)  Indices=1  OutputSizes=1
  Data Store Read8 : DataStoreRead  DataStoreName=RED_IMU_Measurements  IndexOptions=Index vector (dialog)  Indices=1  OutputSizes=1
  Data Store Read83 : DataStoreRead  DataStoreName=BLUE_Control_Law_Enabler  IndexOptions=Index vector (dialog)  Indices=1  OutputSizes=1
  Data Store Read84 : DataStoreRead  DataStoreName=Float_State  IndexOptions=Index vector (dialog)  Indices=1  OutputSizes=1
  Data Store Read85 : DataStoreRead  DataStoreName=WhoAmI  IndexOptions=Index vector (dialog)  Indices=1  OutputSizes=1
  Data Store Read86 : DataStoreRead  DataStoreName=isSim  IndexOptions=Index vector (dialog)  Indices=1  OutputSizes=1
  Data Store Read9 : DataStoreRead  DataStoreName=BLACK_Saturated_Controls  IndexOptions=Index vector (dialog)  Indices=1  OutputSizes=1
  Demux{,1,3..7,9..15,17..18,20..21} (18 alike) : Demux  Outputs=3
  Demux ARM PWM : Demux  Outputs=3
  Demux ARM Status : Demux  Outputs=5
  Demux16 : Demux  Outputs=9
  Demux19 : Demux  Outputs=6
  Demux2 : Demux  Outputs=9
  Demux8 : Demux  Outputs=9
  Read ARM Measured PWM : DataStoreRead  DataStoreName=ARM_Measured_PWM  IndexOptions=Index vector (dialog)  Indices=1  OutputSizes=1
  Read ARM Servo Status : DataStoreRead  DataStoreName=ARM_Servo_Status  IndexOptions=Index vector (dialog)  Indices=1  OutputSizes=1
  To Workspace1 : ToWorkspace  VariableName=dataPacket  SaveFormat=Timeseries  SampleTime=-1
      settings: Save2DSignal=2-D array (concatenate along first dimension)
  wires:
  Data Store Read/1 -> Data Logging Bus/99  "VIS_Measured_States"
  Data Store Read2/1 -> Data Logging Bus/100  "VIS_Confidence"
  Data Logging Bus/1 -> Data Logger/1(Data), To Workspace1/1
  Demux3/1 -> Data Logging Bus/17  "RED_Px_Desired_m"
  Demux19/1 -> Data Logging Bus/32  "ARM_Rz_Shoulder_rad"
  Demux10/1 -> Data Logging Bus/62  "BLACK_IMU_Ax_mpers2"
  Demux2/1 -> Data Logging Bus/8  "RED_Px_m"
  Demux6/1 -> Data Logging Bus/44  "BLACK_Fx_N"
  Demux16/6 -> Data Logging Bus/81  "BLUE_RzD_radpers"
  Demux8/3 -> Data Logging Bus/52  "BLACK_Rz_rad"
  Data Store Read3/1 -> Demux5/1
  Data Store Read1/1 -> Demux1/1
  Demux8/7 -> Data Logging Bus/56  "BLACK_Ax_mpers2"
  Demux2/9 -> Data Logging Bus/16  "RED_RzDD_radpers2"
  Demux12/2 -> Data Logging Bus/89  "BLUE_IMU_Ay_mpers2"
  Demux2/8 -> Data Logging Bus/15  "RED_Ay_mpers2"
  Demux7/1 -> Data Logging Bus/47  "BLACK_Fx_Sat_N"
  Demux13/3 -> Data Logging Bus/95  "BLUE_Rz_Path_rad"
  Data Store Read16/1 -> Demux15/1
  Demux16/5 -> Data Logging Bus/80  "BLUE_Vy_mpers"
  Demux16/2 -> Data Logging Bus/77  "BLUE_Py_m"
  Data Store Read19/1 -> Demux11/1
  Demux21/2 -> Data Logging Bus/42  "ARM_Elbow_Desired"
  Data Store Read9/1 -> Demux7/1
  Data Store Read27/1 -> Data Logging Bus/91  "BLUE_Duty_Cycle"
  Demux14/1 -> Data Logging Bus/70  "BLUE_Fx_N"
  Data Store Read8/1 -> Demux4/1
  Demux5/1 -> Data Logging Bus/25  "RED_Px_Path_m"
  Demux21/3 -> Data Logging Bus/43  "ARM_Wrist_Desired"
  Demux16/4 -> Data Logging Bus/79  "BLUE_Vx_mpers"
  Demux5/3 -> Data Logging Bus/27  "RED_Rz_Path_rad"
  Demux8/6 -> Data Logging Bus/55  "BLACK_RzD_radpers"
  Demux16/9 -> Data Logging Bus/84  "BLUE_RzDD_radpers2"
  Data Store Read85/1 -> Data Logging Bus/97  "Platform_Identification"
  Demux18/1 -> Data Logging Bus/29  "ARM_Shoulder_Command"
  Demux16/1 -> Data Logging Bus/76  "BLUE_Px_m"
  Data Store Read17/1 -> Demux13/1
  Demux8/4 -> Data Logging Bus/53  "BLACK_Vx_mpers"
  Demux8/5 -> Data Logging Bus/54  "BLACK_Vy_mpers"
  Demux5/2 -> Data Logging Bus/26  "RED_Py_Path_m"
  Data Store Read21/1 -> Demux18/1
  Demux3/3 -> Data Logging Bus/19  "RED_Rz_Desired_rad"
  Demux6/2 -> Data Logging Bus/45  "BLACK_Fy_N"
  Data Store Read11/1 -> Demux9/1
  Data Store Read12/1 -> Demux10/1
  Data Store Read60/1 -> Data Logging Bus/66  "BLACK_Control_Law_Enabler"
  Data Store Read84/1 -> Data Logging Bus/96  "Float_State"
  Demux17/1 -> Data Logging Bus/85  "BLUE_Px_Desired_m"
  Data Store Read13/1 -> Demux16/1
  Demux6/3 -> Data Logging Bus/46  "BLACK_Tz_Nm"
  Demux11/3 -> Data Logging Bus/69  "BLACK_Rz_Path_rad"
  Demux20/3 -> Data Logging Bus/40  "ARM_Wrist_Path"
  Data Store Read26/1 -> Data Logging Bus/65  "BLACK_Duty_Cycle"
  Demux15/2 -> Data Logging Bus/74  "BLUE_Fy_Sat_N"
  Demux20/2 -> Data Logging Bus/39  "ARM_Elbow_Path"
  Data Store Read22/1 -> Demux21/1
  Data Store Read23/1 -> Data Logging Bus/28  "ARM_Control_Mode"
  Demux2/6 -> Data Logging Bus/13  "RED_RzD_radpers"
  Data Store Read10/1 -> Demux8/1
  Demux9/1 -> Data Logging Bus/59  "BLACK_Px_Desired_m"
  Demux1/1 -> Data Logging Bus/5  "RED_Fx_Sat_N"
  Demux8/8 -> Data Logging Bus/57  "BLACK_Ay_mpers2"
  Data Store Read6/1 -> Demux2/1
  Demux2/7 -> Data Logging Bus/14  "RED_Ax_mpers2"
  Data Store Read5/1 -> Demux/1
  Demux12/3 -> Data Logging Bus/90  "BLUE_IMU_Gz_radpers"
  Demux19/6 -> Data Logging Bus/37  "ARM_RzD_Wrist_radpers"
  Data Store Read18/1 -> Demux14/1
  Demux14/2 -> Data Logging Bus/71  "BLUE_Fy_N"
  Demux10/2 -> Data Logging Bus/63  "BLACK_IMU_Ay_mpers2"
  Demux/1 -> Data Logging Bus/2  "RED_Fx_N"
  Data Store Read30/1 -> Demux20/1
  Demux11/2 -> Data Logging Bus/68  "BLACK_Py_Path_m"
  Demux13/2 -> Data Logging Bus/94  "BLUE_Py_Path_m"
  Data Store Read24/1 -> Demux6/1
  Demux2/5 -> Data Logging Bus/12  "RED_Vy_mpers"
  Demux2/4 -> Data Logging Bus/11  "RED_Vx_mpers"
  Demux14/3 -> Data Logging Bus/72  "BLUE_Tz_Nm"
  Demux16/7 -> Data Logging Bus/82  "BLUE_Ax_mpers2"
  Demux4/1 -> Data Logging Bus/20  "RED_IMU_Ax_mpers2"
  Demux7/2 -> Data Logging Bus/48  "BLACK_Fy_Sat_N"
  Demux4/3 -> Data Logging Bus/22  "RED_IMU_Gz_radpers"
  Demux16/8 -> Data Logging Bus/83  "BLUE_Ay_mpers2"
  Demux8/9 -> Data Logging Bus/58  "BLACK_RzDD_radpers2"
  Data Store Read83/1 -> Data Logging Bus/92  "BLUE_Control_Law_Enabler"
  Demux16/3 -> Data Logging Bus/78  "BLUE_Rz_rad"
  Demux4/2 -> Data Logging Bus/21  "RED_IMU_Ay_mpers2"
  Demux7/3 -> Data Logging Bus/49  "BLACK_Tz_Sat_Nm"
  Demux1/2 -> Data Logging Bus/6  "RED_Fy_Sat_N"
  Demux19/2 -> Data Logging Bus/33  "ARM_Rz_Elbow_rad"
  Demux13/1 -> Data Logging Bus/93  "BLUE_Px_Path_m"
  Data Store Read14/1 -> Demux17/1
  Demux10/3 -> Data Logging Bus/64  "BLACK_IMU_Gz_radpers"
  Data Store Read37/1 -> Data Logging Bus/24  "RED_Control_Law_Enabler"
  Data Store Read86/1 -> Data Logging Bus/98  "Simulation_Flag"
  Demux19/4 -> Data Logging Bus/35  "ARM_RzD_Shoulder_radpers"
  Demux11/1 -> Data Logging Bus/67  "BLACK_Px_Path_m"
  Demux18/2 -> Data Logging Bus/30  "ARM_Elbow_Command"
  Demux15/1 -> Data Logging Bus/73  "BLUE_Fx_Sat_N"
  Demux17/2 -> Data Logging Bus/86  "BLUE_Py_Desired_m"
  Demux19/3 -> Data Logging Bus/34  "ARM_Rz_Wrist_rad"
  Data Store Read15/1 -> Demux12/1
  Demux1/3 -> Data Logging Bus/7  "RED_Tz_Sat_Nm"
  Demux9/3 -> Data Logging Bus/61  "BLACK_Rz_Desired_rad"
  Demux/2 -> Data Logging Bus/3  "RED_Fy_N"
  Demux3/2 -> Data Logging Bus/18  "RED_Py_Desired_m"
  Demux15/3 -> Data Logging Bus/75  "BLUE_Tz_Sat_Nm"
  Demux2/2 -> Data Logging Bus/9  "RED_Py_m"
  Data Store Read7/1 -> Demux3/1
  Demux20/1 -> Data Logging Bus/38  "ARM_Shoulder_Path"
  Data Store Read4/1 -> Data Logging Bus/1  "Time_s"
  Demux2/3 -> Data Logging Bus/10  "RED_Rz_rad"
  Demux8/2 -> Data Logging Bus/51  "BLACK_Py_m"
  Demux8/1 -> Data Logging Bus/50  "BLACK_Px_m"
  Data Store Read20/1 -> Demux19/1
  Demux17/3 -> Data Logging Bus/87  "BLUE_Rz_Desired_rad"
  Demux21/1 -> Data Logging Bus/41  "ARM_Shoulder_Desired"
  Data Store Read25/1 -> Data Logging Bus/23  "RED_Duty_Cycle"
  Demux12/1 -> Data Logging Bus/88  "BLUE_IMU_Ax_mpers2"
  Demux19/5 -> Data Logging Bus/36  "ARM_RzD_Elbow_radpers"
  Demux9/2 -> Data Logging Bus/60  "BLACK_Py_Desired_m"
  Demux18/3 -> Data Logging Bus/31  "ARM_Wrist_Command"
  Demux/3 -> Data Logging Bus/4  "RED_Tz_Nm"
  Read ARM Measured PWM/1 -> Demux ARM PWM/1
  Read ARM Servo Status/1 -> Demux ARM Status/1
  Demux ARM PWM/1 -> Data Logging Bus/101  "ARM_Shoulder_PWM"
  Demux ARM PWM/2 -> Data Logging Bus/102  "ARM_Elbow_PWM"
  Demux ARM PWM/3 -> Data Logging Bus/103  "ARM_Wrist_PWM"
  Demux ARM Status/1 -> Data Logging Bus/104  "ARM_Servos_Read"
  Demux ARM Status/2 -> Data Logging Bus/105  "ARM_Servo_Read_ms"
  Demux ARM Status/3 -> Data Logging Bus/106  "ARM_USB_Latency_ms"
  Demux ARM Status/4 -> Data Logging Bus/107  "ARM_Servo_Reads_Missed"
  Demux ARM Status/5 -> Data Logging Bus/108  "ARM_Servo_Alert"

== system Template_v5_0_0_2026a_Original/Debugger ==
  BLACK_Logger text : StringToASCII  OutputVectorSize=120
  BLUE_Logger text : StringToASCII  OutputVectorSize=120
  Data Store Read : DataStoreRead  DataStoreName=RED_Logger  IndexOptions=Index vector (dialog)  Indices=1  OutputSizes=1
  Data Store Read2 : DataStoreRead  DataStoreName=BLACK_Logger  IndexOptions=Index vector (dialog)  Indices=1  OutputSizes=1
  Data Store Read3 : DataStoreRead  DataStoreName=BLUE_Logger  IndexOptions=Index vector (dialog)  Indices=1  OutputSizes=1
  RED_Logger text : StringToASCII  OutputVectorSize=120
  Send Debug Messages : MATLAB Function  TreatAsAtomicUnit=on
  Univ_Time : DataStoreRead  DataStoreName=Univ_Time  IndexOptions=Index vector (dialog)  Indices=1  OutputSizes=1
  WhoAmI : DataStoreRead  DataStoreName=WhoAmI  IndexOptions=Index vector (dialog)  Indices=1  OutputSizes=1
  isSim : DataStoreRead  DataStoreName=isSim  IndexOptions=Index vector (dialog)  Indices=1  OutputSizes=1
  wires:
  Data Store Read/1 -> RED_Logger text/1
  Data Store Read2/1 -> BLACK_Logger text/1
  Data Store Read3/1 -> BLUE_Logger text/1
  WhoAmI/1 -> Send Debug Messages/1(whoAmI)
  isSim/1 -> Send Debug Messages/2(isSim)
  Univ_Time/1 -> Send Debug Messages/3(t)
  RED_Logger text/1 -> Send Debug Messages/4(red)
  BLACK_Logger text/1 -> Send Debug Messages/5(black)
  BLUE_Logger text/1 -> Send Debug Messages/6(blue)
